simulink model "force_position_step4"  (R2025b)
settings: Solver=VariableStepAuto  StartTime=0.0  StopTime=1  RelTol=1e-3
values from neighbouring files (symbols this model uses):
  lut_i_mA = interp1(z_anchor_um, i_anchor_mA, lut_z_um, 'pchip')    [init_force_position_sim_step2.m]
  lut_z_um = linspace(min(z_anchor_um), max(z_anchor_um), 501)    [init_force_position_sim_step2.m]
settings Model: Creator=HYB  LastModifiedBy=HYB

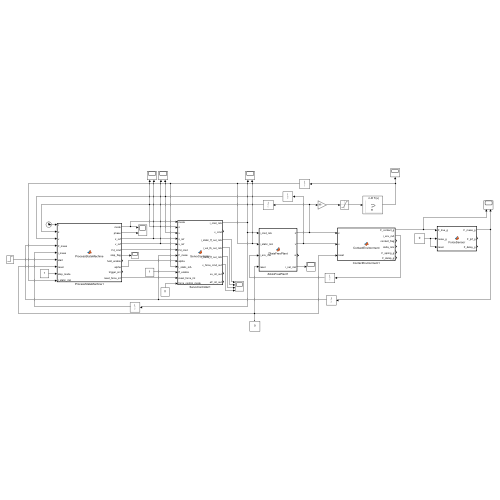
[thumbnail: Simulink's stored preview of the top-level diagram]
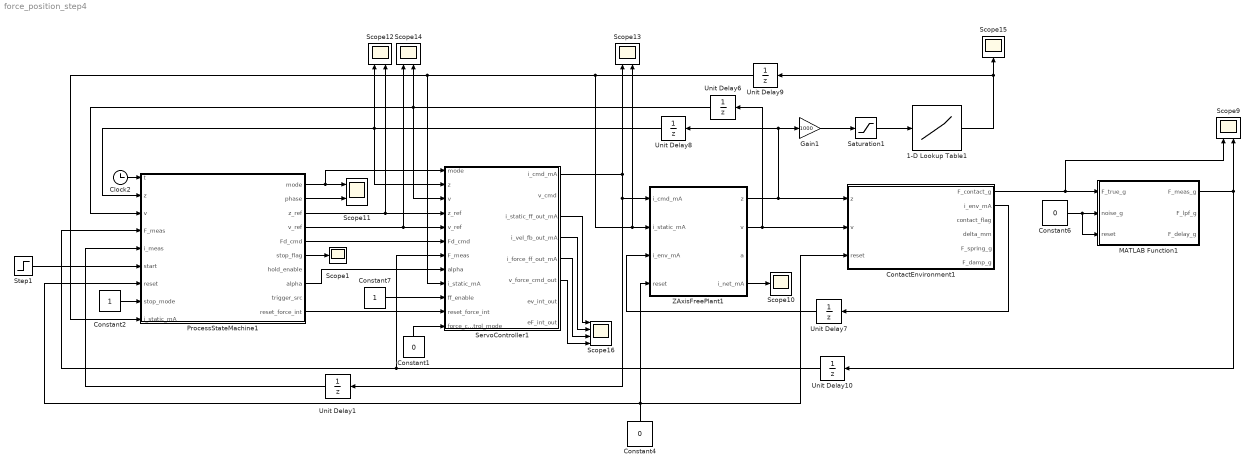
== system force_position_step4 ==
  1-D Lookup Table1 : Lookup_n-D  NumberOfTableDimensions=1  BreakpointsForDimension1=lut_z_um  Table=lut_i_mA  InternalRulePriority=Speed  RndMeth=Simplest
  Clock2 : Clock
  Constant1 : Constant  Value=0
  Constant2 : Constant
  Constant4 : Constant  Value=0
  Constant6 : Constant  Value=0
  Constant7 : Constant
  ContactEnvironment1 : MATLAB Function  TreatAsAtomicUnit=on
  Gain1 : Gain  Gain=1000
  MATLAB Function1 : MATLAB Function  TreatAsAtomicUnit=on
  ProcessStateMachine1 : MATLAB Function  TreatAsAtomicUnit=on
  Saturation1 : Saturate  UpperLimit=15000  LowerLimit=0
  Scope1 : Scope
      settings: ActiveDisplayYMinimum=-0.037280701754385914  ActiveDisplayYMaximum=0.26347117794486219
  Scope10 : Scope
      settings: ActiveDisplayYMinimum=-1967.6933461484089  ActiveDisplayYMaximum=1895.5357153815362  DataLoggingVariableName=ScopeData8
  Scope{9,11..14} (5 alike) : Scope  NumInputPorts=2
      Scope11 settings: ActiveDisplayYMinimum=-0.49999999999999989  ActiveDisplayYMaximum=4.5  DataLoggingVariableName=ScopeData9
      Scope12 settings: ActiveDisplayYMinimum=-1.8525354305786921  ActiveDisplayYMaximum=16.672818875208232  DataLoggingVariableName=ScopeData10
      Scope13 settings: ActiveDisplayYMinimum=-4131.8650549204458  ActiveDisplayYMaximum=3168.7810672371484  DataLoggingVariableName=ScopeData11
      Scope14 settings: ActiveDisplayYMinimum=-0.18374777513732909  ActiveDisplayYMaximum=0.32105225426370021  DataLoggingVariableName=ScopeData12
      Scope9 settings: ActiveDisplayYMinimum=-87.952638061942039  ActiveDisplayYMaximum=791.57374255747845  DataLoggingVariableName=ScopeData15
  Scope15 : Scope
      settings: ActiveDisplayYMinimum=800.135408652136  ActiveDisplayYMaximum=882.66437213169263  DataLoggingVariableName=ScopeData13
  Scope16 : Scope  NumInputPorts=4
      settings: ActiveDisplayYMinimum=-1223.7721714781019  ActiveDisplayYMaximum=889.1636178608212  DataLoggingVariableName=ScopeData14
  ServoController1 : MATLAB Function  TreatAsAtomicUnit=on
  Step1 : Step  Time=0.01  SampleTime=0
  Unit Delay{1,6..10} (6 alike) : UnitDelay  SampleTime=0.001  HasFrameUpgradeWarning=on
  ZAxisFreePlant1 : MATLAB Function  TreatAsAtomicUnit=on
  wires:
  Constant4/1 -> ZAxisFreePlant1/4(reset), ContactEnvironment1/3(reset), ProcessStateMachine1/7(reset)
  ZAxisFreePlant1/2(v) -> Unit Delay6/1, ContactEnvironment1/2(v)
  Unit Delay10/1 -> ServoController1/7(F_meas), ProcessStateMachine1/4(F_meas)
  ProcessStateMachine1/8(alpha) -> ServoController1/8(alpha)
  ZAxisFreePlant1/1(z) -> Gain1/1, Unit Delay8/1, ContactEnvironment1/1(z)
  ProcessStateMachine1/4(v_ref) -> Scope14/1, ServoController1/5(v_ref)
  Unit Delay6/1 -> ServoController1/3(v), ProcessStateMachine1/3(v), Scope14/2
  ContactEnvironment1/2(i_env_mA) -> Unit Delay7/1
  Saturation1/1 -> 1-D Lookup Table1/1
  Unit Delay9/1 -> ZAxisFreePlant1/2(i_static_mA), Scope13/2, ServoController1/9(i_static_mA), ProcessStateMachine1/9(i_static_mA)
  ProcessStateMachine1/5(Fd_cmd) -> ServoController1/6(Fd_cmd)
  ServoController1/6(v_force_cmd_out) -> Scope16/4
  ProcessStateMachine1/2(phase) -> Scope11/2
  Unit Delay8/1 -> ServoController1/2(z), ProcessStateMachine1/2(z), Scope12/1
  Constant7/1 -> ServoController1/10(ff_enable)
  ProcessStateMachine1/3(z_ref) -> Scope12/2, ServoController1/4(z_ref)
  1-D Lookup Table1/1 -> Scope15/1, Unit Delay9/1
  Step1/1 -> ProcessStateMachine1/6(start)
  ServoController1/4(i_vel_fb_out_mA) -> Scope16/2
  Gain1/1 -> Saturation1/1
  ZAxisFreePlant1/4(i_net_mA) -> Scope10/1
  ContactEnvironment1/1(F_contact_g) -> MATLAB Function1/1(F_true_g), Scope9/1
  Unit Delay7/1 -> ZAxisFreePlant1/3(i_env_mA)
  ServoController1/1(i_cmd_mA) -> Unit Delay1/1, ZAxisFreePlant1/1(i_cmd_mA), Scope13/1
  MATLAB Function1/1(F_meas_g) -> Scope9/2, Unit Delay10/1
  Constant6/1 -> MATLAB Function1/2(noise_g), MATLAB Function1/3(reset)
  Clock2/1 -> ProcessStateMachine1/1(t)
  ServoController1/5(i_force_ff_out_mA) -> Scope16/3
  ProcessStateMachine1/10(reset_force_int) -> ServoController1/11(reset_force_int)
  ServoController1/3(i_static_ff_out_mA) -> Scope16/1
  ProcessStateMachine1/1(mode) -> ServoController1/1(mode), Scope11/1
  Constant1/1 -> ServoController1/12(force_control_mode)
  Constant2/1 -> ProcessStateMachine1/8(stop_mode)
  Unit Delay1/1 -> ProcessStateMachine1/5(i_meas)
  ProcessStateMachine1/6(stop_flag) -> Scope1/1

== matlab function force_position_step4/ContactEnvironment1 ==
  data: z input; F_contact_g output; v input; reset input; i_env_mA output; contact_flag output; delta_mm output; F_spring_g output; F_damp_g output
function [F_contact_g, i_env_mA, contact_flag, delta_mm, F_spring_g, F_damp_g] = ContactEnvironment(z, v, reset)
%#codegen

z_contact = 14.30;       % mm

Ke_g_per_mm = 500.0;    % g/mm
Be_g_per_mmps = 2.0;    % g/(mm/s)

F_max_g = 3000.0;
Kforce_mA_per_g = 2.38;

delta = z - z_contact;

if delta <= 0
    delta_mm = 0.0;
    F_spring_g = 0.0;
    F_damp_g = 0.0;
    F_contact_g = 0.0;
    contact_flag = false;
else
    delta_mm = delta;
    contact_flag = true;

    F_spring_g = Ke_g_per_mm * delta_mm;

    % 只在继续向下压入时产生正阻尼力
    if v > 0
        F_damp_g = Be_g_per_mmps * v;
    else
        F_damp_g = 0.0;
    end

    F_contact_g = F_spring_g + F_damp_g;

    if F_contact_g > F_max_g
        F_contact_g = F_max_g;
    end
end

i_env_mA = Kforce_mA_per_g * F_contact_g;

== matlab function force_position_step4/MATLAB Function1 ==
  data: F_true_g input; F_meas_g output; noise_g input; reset input; F_lpf_g output; F_delay_g output
function [F_meas_g, F_lpf_g, F_delay_g] = ForceSensor(F_true_g, noise_g, reset)
%#codegen

% ============================================================
% ForceSensor
%
% 作用：
%   将真实接触力 F_true_g 转换为控制器可见的测量力 F_meas_g。
%
% 模型包含：
%   1. 传感器量程限幅
%   2. 一阶低通滤波
%   3. 采样/传输延迟
%   4. 零偏和噪声
%
% 注意：
%   这个模块只用于测量反馈；
%   环境反力 i_env_mA 不应经过该模块再作用到 ZAxisFreePlant。
% ============================================================

%% 参数
Ts = 1e-3;              % s
tau_sensor = 0.005;     % s，传感器/滤波时间常数
F_sensor_max = 3000.0;  % g，传感器量程上限
F_sensor_min = 0.0;     % g，压缩力为正，第一版不考虑拉力

F_bias = 0.0;           % g，零偏

% 延迟采样点数
% 这里固定为 3，对应 3 ms
N_delay = 3;

%% 一阶低通系数
alpha = exp(-Ts / tau_sensor);

%% 持久变量
persistent y_lpf delay_buf initialized

if isempty(initialized)
    y_lpf = 0.0;
    delay_buf = zeros(1, N_delay);
    initialized = true;
end

if reset
    y_lpf = 0.0;
    delay_buf = zeros(1, N_delay);
end

%% 1. 量程限幅
F_sat = F_true_g;

if F_sat > F_sensor_max
    F_sat = F_sensor_max;
elseif F_sat < F_sensor_min
    F_sat = F_sensor_min;
end

%% 2. 一阶低通滤波
y_lpf = alpha * y_lpf + (1.0 - alpha) * F_sat;
F_lpf_g = y_lpf;

%% 3. 整数采样延迟
% delay_buf(1) 是最旧值，delay_buf(end) 是最新值
F_delay_g = delay_buf(1);

for k = 1:N_delay-1
    delay_buf(k) = delay_buf(k+1);
end
delay_buf(N_delay) = F_lpf_g;

%% 4. 加零偏和噪声
F_meas_g = F_delay_g + F_bias + noise_g;

%% 5. 测量值再次限幅
if F_meas_g > F_sensor_max
    F_meas_g = F_sensor_max;
elseif F_meas_g < F_sensor_min
    F_meas_g = F_sensor_min;
end

== matlab function force_position_step4/ProcessStateMachine1 ==
  data: t input; mode output; z input; v input; F_meas input; i_meas input; start input; reset input; phase output; z_ref output; v_ref output; Fd_cmd output; stop_flag output; hold_enable output; alpha output; trigger_src output; reset_force_int output; stop_mode input; i_static_mA input
function [mode, phase, z_ref, v_ref, Fd_cmd, stop_flag, hold_enable, alpha, trigger_src, reset_force_int] = ...
    ProcessStateMachine(t, z, v, F_meas, i_meas, start, reset, stop_mode, i_static_mA)
%#codegen

% ============================================================
% 力位控制工艺流程状态机
%
% 阶段：
% 0 Ready
% 1 FastPosition: 位置模式快进到 13 mm
% 2 FirstVelocity: 第一速度到 14 mm
% 3 SearchVelocity: 第二速度搜索接触
% 4 ForceHold: 力控/保压模式
% 5 ErrorStop: 超行程或异常停止
%
% stop_mode 判停方式：
% 1：压力判停
% 2：速度判停
% 3：电流残差判停
% 4：速度 + 压力判停
% 5：速度 + 电流残差判停
%
% 电流残差：
% i_res = i_meas - i_static_mA
%
% 说明：
% i_meas 可以接实际电机电流、驱动器反馈电流，仿真中也可以先接 i_cmd_mA。
% i_static_mA 接静态 PCHIP 查表输出。
% ============================================================


%% ---------- 可调参数 ----------
z_fast_end = 13.0;     % mm
z_v1_end   = 14.0;     % mm
z_max      = 15.0;     % mm

pos_tol = 0.02;        % mm

v1_search = 5.0;       % mm/s
v2_search = 1.0;       % mm/s

%% 压力判停参数
F_th = 10.0;                 % g
T_force_confirm = 0.001;     % s

%% 速度判停参数
v_stop_th = 0.1;            % mm/s
T_v_confirm = 0.005;         % s

%% 电流残差判停参数
% 注意：
% 这里不再使用原始 i_meas 阈值，而是使用：
% i_res = i_meas - i_static_mA
%
% 阈值需要根据仿真或真实实验调整。
% 如果 i_res 是总电流扣除静态项，里面还包含速度环动态电流、摩擦电流，
% 阈值不宜太小。
i_res_stop_th = 20.0;       % mA，示例值，需要根据数据调整
T_i_confirm = 0.003;         % s

% 电流残差判停是否取绝对值
% true ：abs(i_res) > 阈值
% false：i_res > 阈值
%
% 如果接触后电流残差一定正向增加，可以设为 false；
% 如果存在方向、回弹或控制器反向电流，建议 true。
use_abs_i_res = true;

%% 目标保压力
Fd_set = 200.0;             % g
T_ramp_force = 0.010;        % s


%% ---------- 状态变量 ----------
persistent state t_enter tF_start tV_start tI_start prev_state last_trigger_src

if isempty(state)
    state = int32(0);
    prev_state = int32(0);
    t_enter = 0.0;
    tF_start = -1.0;
    tV_start = -1.0;
    tI_start = -1.0;
    last_trigger_src = 0;
end

if reset
    state = int32(0);
    prev_state = int32(0);
    t_enter = t;
    tF_start = -1.0;
    tV_start = -1.0;
    tI_start = -1.0;
    last_trigger_src = 0;
end


%% ---------- 默认输出 ----------
mode = 0;
phase = double(state);

% 默认保持当前位置，避免模式切换瞬间目标突变
z_ref = z;
v_ref = 0.0;

Fd_cmd = Fd_set;

stop_flag = false;
hold_enable = false;

% alpha 在保压阶段从 0 平滑到 1
alpha = 0.0;

% trigger_src:
% 0 none
% 1 force
% 2 velocity
% 3 current residual
% 4 z_max
% 5 velocity + force
% 6 velocity + current residual
trigger_src = last_trigger_src;

reset_force_int = false;

prev_state = state;


%% ---------- 启动逻辑 ----------
if state == 0
    mode = 0;
    phase = 0;
    z_ref = z;
    v_ref = 0.0;
    alpha = 0.0;
    
    if start
        state = int32(1);
        t_enter = t;
        last_trigger_src = 0;
    end
end


%% ---------- 状态 1：位置快进 ----------
if state == 1
    mode = 1;
    phase = 1;
    z_ref = z_fast_end;
    v_ref = 0.0;
    alpha = 0.0;
    
    if z >= z_fast_end - pos_tol
        state = int32(2);
        t_enter = t;
    end
end


%% ---------- 状态 2：第一速度 ----------
if state == 2
    mode = 2;          % 速度模式
    phase = 2;
    z_ref = z;
    v_ref = v1_search;
    alpha = 0.0;
    
    if z >= z_v1_end - pos_tol
        state = int32(3);
        t_enter = t;
        
        % 进入搜索阶段时，清空各判停计时
        tF_start = -1.0;
        tV_start = -1.0;
        tI_start = -1.0;
    end
end


%% ---------- 状态 3：第二速度搜索 ----------
if state == 3
    mode = 2;          % 速度模式
    phase = 3;
    z_ref = z;
    v_ref = v2_search;
    alpha = 0.0;
    
    %% ========================================================
    % 1. 压力条件 force_ok
    % =========================================================
    if F_meas > F_th
        if tF_start < 0.0
            tF_start = t;
        end
    else
        tF_start = -1.0;
    end
    
    force_ok = false;
    if tF_start >= 0.0
        if (t - tF_start) >= T_force_confirm
            force_ok = true;
        end
    end
    
    
    %% ========================================================
    % 2. 速度条件 velocity_ok
    % =========================================================
    if abs(v) < v_stop_th
        if tV_start < 0.0
            tV_start = t;
        end
    else
        tV_start = -1.0;
    end
    
    velocity_ok = false;
    if tV_start >= 0.0
        if (t - tV_start) >= T_v_confirm
            velocity_ok = true;
        end
    end
    
    
    %% ========================================================
    % 3. 电流残差条件 current_ok
    %
    % 原始电流判停：
    %     abs(i_meas) > i_stop_th
    %
    % 修改后：
    %     i_res = i_meas - i_static_mA
    %
    % 这样能够扣除位置相关静态负载电流。
    % =========================================================
    i_res = i_meas - i_static_mA;
    
    if use_abs_i_res
        current_condition = abs(i_res) > i_res_stop_th;
    else
        current_condition = i_res > i_res_stop_th;
    end
    
    if current_condition
        if tI_start < 0.0
            tI_start = t;
        end
    else
        tI_start = -1.0;
    end
    
    current_ok = false;
    if tI_start >= 0.0
        if (t - tI_start) >= T_i_confirm
            current_ok = true;
        end
    end
    
    
    %% ========================================================
    % 4. 根据 stop_mode 选择判停方式
    % =========================================================
    stop_condition = false;
    selected_trigger = 0;
    
    if stop_mode < 1.5
        %% 1：压力判停
        if force_ok
            stop_condition = true;
            selected_trigger = 1;
        end
        
    elseif stop_mode < 2.5
        %% 2：速度判停
        if velocity_ok
            stop_condition = true;
            selected_trigger = 2;
        end
        
    elseif stop_mode < 3.5
        %% 3：电流残差判停
        if current_ok
            stop_condition = true;
            selected_trigger = 3;
        end
        
    elseif stop_mode < 4.5
        %% 4：速度 + 压力判停
        if velocity_ok && force_ok
            stop_condition = true;
            selected_trigger = 5;
        end
        
    elseif stop_mode < 5.5
        %% 5：速度 + 电流残差判停
        if velocity_ok && current_ok
            stop_condition = true;
            selected_trigger = 6;
        end
        
    else
        %% 输入异常时，默认压力判停
        if force_ok
            stop_condition = true;
            selected_trigger = 1;
        end
    end
    
    
    %% ========================================================
    % 5. 执行停止或安全保护
    % =========================================================
    if stop_condition
        state = int32(4);
        t_enter = t;
        last_trigger_src = selected_trigger;
        trigger_src = selected_trigger;
        stop_flag = true;
        
    elseif z >= z_max
        state = int32(5);
        t_enter = t;
        last_trigger_src = 4;
        trigger_src = 4;
    end
end


%% ---------- 状态 4：力控 / 保压 ----------
if state == 4
    mode = 3;          % 力控 / 保压模式
    phase = 4;
    z_ref = z;
    v_ref = 0.0;
    Fd_cmd = Fd_set;
    stop_flag = true;
    hold_enable = true;
    
    % 目标力前馈平滑引入系数 alpha: 0 -> 1
    tau = (t - t_enter) / T_ramp_force;
    if tau < 0.0
        tau = 0.0;
    elseif tau > 1.0
        tau = 1.0;
    end
    
    % S型平滑
    alpha = 3.0 * tau * tau - 2.0 * tau * tau * tau;
end


%% ---------- 状态 5：安全停止 ----------
if state == 5
    mode = 9;
    phase = 5;
    z_ref = z;
    v_ref = 0.0;
    Fd_cmd = 0.0;
    stop_flag = true;
    hold_enable = false;
    alpha = 0.0;
end


%% ---------- 进入保压瞬间复位力控积分 ----------
if prev_state ~= int32(4) && state == int32(4)
    reset_force_int = true;
else
    reset_force_int = false;
end

phase = double(state);

end

== matlab function force_position_step4/ServoController1 ==
  data: mode input; i_cmd_mA output; z input; v input; z_ref input; v_ref input; Fd_cmd input; F_meas input; alpha input; i_static_mA input; ff_enable input; reset_force_int input; v_cmd output; i_static_ff_out_mA output; i_vel_fb_out_mA output; i_force_ff_out_mA output; v_force_cmd_out output; ev_int_out output; eF_int_out output; force_control_mode input
function [i_cmd_mA, v_cmd, i_static_ff_out_mA, i_vel_fb_out_mA, ...
          i_force_ff_out_mA, v_force_cmd_out, ev_int_out, eF_int_out] = ...
    ServoController(mode, z, v, z_ref, v_ref, Fd_cmd, F_meas, alpha, ...
                    i_static_mA, ff_enable, reset_force_int, force_control_mode)
%#codegen

% ============================================================
% ServoController
%
% mode = 1：位置模式
%   位置外环 -> 速度PI -> 电流
%
% mode = 2：速度模式
%   速度指令 -> 速度PI -> 电流
%
% mode = 3：保压/力控模式
%   force_control_mode = 0：开环力控
%       i_cmd = i_static_ff + i_force_ff
%
%   force_control_mode = 1：闭环力控
%       力外环 -> 速度指令 -> 速度PI -> 电流
%       保留原来的闭环算法逻辑
%
% mode = 9：安全停止
%
% 下行方向为正：
%   z 增大表示压头向下
%   v > 0 表示继续下压
%   F_meas 为压缩力，单位 g
% ============================================================

%% ============================================================
% 1. 基本参数
% ============================================================

Ts = 1e-3;              % 控制周期，s

%% 位置环参数
Kp_pos = 100.0;         % (mm/s)/mm
v_fast_max = 100.0;     % mm/s

%% 速度内环 PI 参数
Kvp = 20.0;             % mA/(mm/s)
Kvi = 200.0;            % mA/mm

i_vel_int_limit = 3000.0;   % 速度积分项对应电流限幅，mA

%% 力外环参数：力误差 -> 速度指令
% eF > 0 表示实际力小于目标力，需要继续下压，v_cmd > 0
% eF < 0 表示实际力超过目标力，需要回退，v_cmd < 0

Kfp_v_per_g = 0.05;       % (mm/s)/g
Kfi_v_per_gs = 0.5;       % (mm/s)/(g*s)

v_force_limit = 5.0;      % 闭环力控阶段最大速度，mm/s
v_force_int_limit = 3.0;  % 力积分产生的速度限幅，mm/s

%% 目标力电流前馈
% 闭环模式下是否保留目标力电流前馈
% 0：严格力环 -> 速度环
% 1：复合控制，目标力电流前馈 + 力环速度修正
force_current_ff_enable = 1.0;

% 开环模式下一定会使用这个系数
Kforce_mA_per_g = 2.38;    % mA/g

%% 总电流限幅
i_limit = 4500.0;         % mA，即 5 A

%% ============================================================
% 2. 持久变量
% ============================================================

persistent ev_int eF_int last_mode

if isempty(ev_int)
    ev_int = 0.0;
    eF_int = 0.0;
    last_mode = 0.0;
end

%% ============================================================
% 3. 模式切换处理
% ============================================================

% 进入保压时，复位力积分
if reset_force_int
    eF_int = 0.0;
end

% 从位置/速度模式切入力控模式时，清掉速度积分
% 避免切换前的速度环积分继续影响保压阶段
if last_mode ~= 3 && mode == 3
    ev_int = 0.0;
end

% 安全停止时清空积分
if mode == 9
    ev_int = 0.0;
    eF_int = 0.0;
end

%% ============================================================
% 4. 默认输出
% ============================================================

v_cmd = 0.0;
v_force_cmd = 0.0;

i_static_ff_mA = 0.0;
i_vel_fb_mA = 0.0;
i_force_ff_mA = 0.0;

% 是否启用速度 PI 内环
use_speed_loop = false;

%% ============================================================
% 5. 静态前馈
% ============================================================

if ff_enable > 0.5
    i_static_ff_mA = i_static_mA;
else
    i_static_ff_mA = 0.0;
end

%% ============================================================
% 6. 生成速度指令或开环电流
% ============================================================

if mode == 1
    %% --------------------------------------------------------
    % 位置模式：位置外环输出速度指令
    % ---------------------------------------------------------
    
    e_pos = z_ref - z;
    v_cmd = Kp_pos * e_pos;
    
    if v_cmd > v_fast_max
        v_cmd = v_fast_max;
    elseif v_cmd < -v_fast_max
        v_cmd = -v_fast_max;
    end
    
    use_speed_loop = true;
    
elseif mode == 2
    %% --------------------------------------------------------
    % 速度模式：直接使用状态机给出的速度指令
    % ---------------------------------------------------------
    
    v_cmd = v_ref;
    use_speed_loop = true;
    
elseif mode == 3
    %% --------------------------------------------------------
    % 保压 / 力控模式
    %
    % force_control_mode = 0：开环力控
    % force_control_mode = 1：闭环力控，力环 -> 速度环
    % ---------------------------------------------------------
    
    % 目标力平滑引入
    F_ref = alpha * Fd_cmd;
    
    if force_control_mode < 0.5
        %% ----------------------------------------------------
        % 开环力控
        %
        % 不使用 F_meas 修正；
        % 不使用速度环；
        % 只输出：静态前馈 + 目标力电流前馈。
        % -----------------------------------------------------
        
        v_cmd = 0.0;
        v_force_cmd = 0.0;
        use_speed_loop = false;
        
        % 开环目标力电流前馈
        i_force_ff_mA = Kforce_mA_per_g * F_ref;
        
        % 开环模式下不更新力积分，避免切回闭环时残留
        eF_int = 0.0;
        
        % 开环模式下速度积分也清零，避免前一阶段残留
        ev_int = 0.0;
        
    else
        %% ----------------------------------------------------
        % 闭环力控：力外环 -> 速度指令 -> 速度 PI -> 电流
        %
        % 这一部分保持你原有闭环算法逻辑。
        % -----------------------------------------------------
        
        % 力误差
        eF = F_ref - F_meas;
        
        % 力积分
        eF_int = eF_int + eF * Ts;
        
        % 力积分转速度
        vF_i = Kfi_v_per_gs * eF_int;
        
        % 力积分限幅
        if vF_i > v_force_int_limit
            vF_i = v_force_int_limit;
            eF_int = vF_i / Kfi_v_per_gs;
        elseif vF_i < -v_force_int_limit
            vF_i = -v_force_int_limit;
            eF_int = vF_i / Kfi_v_per_gs;
        end
        
        % 力比例项转速度
        vF_p = Kfp_v_per_g * eF;
        
        % 力外环输出速度指令
        v_force_cmd = vF_p + vF_i;
        
        % 力控阶段速度限幅
        if v_force_cmd > v_force_limit
            v_force_cmd = v_force_limit;
        elseif v_force_cmd < -v_force_limit
            v_force_cmd = -v_force_limit;
        end
        
        v_cmd = v_force_cmd;
        use_speed_loop = true;
        
        % 可选目标力电流前馈
        if force_current_ff_enable > 0.5
            i_force_ff_mA = Kforce_mA_per_g * F_ref;
        else
            i_force_ff_mA = 0.0;
        end
    end
    
elseif mode == 9
    %% --------------------------------------------------------
    % 安全停止
    % ---------------------------------------------------------
    
    v_cmd = 0.0;
    v_force_cmd = 0.0;
    
    i_static_ff_mA = 0.0;
    i_force_ff_mA = 0.0;
    
    use_speed_loop = false;
    
else
    %% --------------------------------------------------------
    % Ready / Off
    % ---------------------------------------------------------
    
    v_cmd = 0.0;
    v_force_cmd = 0.0;
    
    i_static_ff_mA = 0.0;
    i_force_ff_mA = 0.0;
    
    use_speed_loop = false;
end

%% ============================================================
% 7. 速度 PI 内环
% ============================================================

if use_speed_loop
    
    e_v = v_cmd - v;
    
    % 比例项
    i_v_p = Kvp * e_v;
    
    % 积分项
    ev_int = ev_int + e_v * Ts;
    i_v_i = Kvi * ev_int;
    
    % 速度积分项限幅
    if i_v_i > i_vel_int_limit
        i_v_i = i_vel_int_limit;
        ev_int = i_v_i / Kvi;
    elseif i_v_i < -i_vel_int_limit
        i_v_i = -i_vel_int_limit;
        ev_int = i_v_i / Kvi;
    end
    
    i_vel_fb_mA = i_v_p + i_v_i;
    
else
    i_vel_fb_mA = 0.0;
end

%% ============================================================
% 8. 合成电流
% ============================================================

i_cmd_unsat = i_static_ff_mA ...
            + i_vel_fb_mA ...
            + i_force_ff_mA;

i_cmd_mA = i_cmd_unsat;

%% 总电流限幅
if i_cmd_mA > i_limit
    i_cmd_mA = i_limit;
elseif i_cmd_mA < -i_limit
    i_cmd_mA = -i_limit;
end

%% ============================================================
% 9. 抗积分饱和
% ============================================================

if use_speed_loop
    if i_cmd_unsat ~= i_cmd_mA
        
        e_v_aw = v_cmd - v;
        
        % 如果电流已经正向饱和，而速度误差还要求继续增加正向电流，
        % 则回退速度积分。
        if (i_cmd_unsat > i_limit && e_v_aw > 0.0) || ...
           (i_cmd_unsat < -i_limit && e_v_aw < 0.0)
            ev_int = ev_int - 0.5 * e_v_aw * Ts;
        end
    end
end

% 力外环速度饱和时，也做一点简单抗饱和
% 只在闭环力控模式下启用。
if mode == 3 && force_control_mode >= 0.5
    
    F_ref_aw = alpha * Fd_cmd;
    eF_aw = F_ref_aw - F_meas;
    
    vF_unsat = Kfp_v_per_g * eF_aw + Kfi_v_per_gs * eF_int;
    
    if (vF_unsat > v_force_limit && eF_aw > 0.0) || ...
       (vF_unsat < -v_force_limit && eF_aw < 0.0)
        eF_int = eF_int - 0.5 * eF_aw * Ts;
    end
end

%% ============================================================
% 10. 输出监控量
% ============================================================

i_static_ff_out_mA = i_static_ff_mA;
i_vel_fb_out_mA    = i_vel_fb_mA;
i_force_ff_out_mA  = i_force_ff_mA;

v_force_cmd_out = v_force_cmd;

ev_int_out = ev_int;
eF_int_out = eF_int;

last_mode = mode;

== matlab function force_position_step4/ZAxisFreePlant1 ==
  data: i_cmd_mA input; z output; i_static_mA input; i_env_mA input; reset input; v output; a output; i_net_mA output
function [z, v, a, i_net_mA] = ZAxisFreePlant(i_cmd_mA, i_static_mA, i_env_mA, reset)
%#codegen

% ============================================================
% 简化Z轴自由运动模型
%
% 下行方向为正：
%   z 增大表示压头向下伸出
%
% i_static_mA 是实验一得到的下行静态保持电流。
% 在对象模型中，它作为位置相关的非线性负载项。
%
% 简化模型：
%   a = Kacc * (i_cmd - i_static(z) - Cv*v - Icoul*tanh(v/vs))
% ============================================================

%% 参数
Ts = 1e-3;

z0 = 0.0;          % 初始位置，mm
v0 = 0.0;

z_min = 0.0;
z_max = 40;      % z轴最大行程
v_limit = 1200.0;          % 硬件速度上限mm/s

Kt_N_per_A = 4.12;
M_eff = 0.20;              % kg，先估计
Kacc = Kt_N_per_A / M_eff; % ≈ 20.6 mm/s^2 per mA

Cv_mA = 1.0;       % mA/(mm/s)
Icoul_mA = 2.0;    % mA
vs = 0.05;         % mm/s，tanh平滑速度

persistent z_k v_k

if isempty(z_k)
    z_k = z0;
    v_k = v0;
end

if reset
    z_k = z0;
    v_k = v0;
end

%% 摩擦电流
i_fric_mA = Cv_mA * v_k + Icoul_mA * tanh(v_k / vs);

%% 净驱动电流
i_net_mA = i_cmd_mA - i_static_mA - i_fric_mA - i_env_mA;

%% 加速度
a = Kacc * i_net_mA;

%% 积分
v_k = v_k + Ts * a;
z_k = z_k + Ts * v_k;

%% 行程限位
if z_k < z_min
    z_k = z_min;
    if v_k < 0
        v_k = 0.0;
    end
elseif z_k > z_max
    z_k = z_max;
    if v_k > 0
        v_k = 0.0;
    end
end

z = z_k;
v = v_k;
